simulink model "Controller_damping_cbf_22Franka"  (R2022b)
settings: Solver=FixedStepDiscrete  StartTime=0.0  StopTime=inf  FixedStep=0.001  RelTol=1e-3
PreLoadFcn:
  | set_param(gcs, 'RTWSystemTargetFile', 'franka_emika_panda.tlc');
  | 
  | demos_common_configs();
  | collision_behavior = ones(1,52)*100;
values from neighbouring files (symbols this model uses):
  b_sg = fliplr(B(end, :))    [init_damping_cbf.m]
  cbf_damping_params = [cbf_p_ths; cbf_v_ths; cbf_v_0; cbf_gamma; cbf_d_max;                        cbf_w_lin; cbf_w_quad; plane_normal; plane_offset;                        cbf_latch_entry; cbf_zone_hyst; cbf_latch_alpha; cbf_clip_drift;                        cbf_tau_rate; cbf_dt; cbf_gamma_pos_scale]    [init_damping_cbf.m]
  cbf_kappa = 0.85 * cbf_d_max / cbf_rho_eff    (= 82.6388888889)    [init_damping_cbf.m]
  cbf_stiff_decouple = 0    [init_damping_cbf.m]
  Dn = 20 * ones(7,1)    [init_damping_cbf.m]
  H_home = getTransform(Franka_robot, q_home, 'panda_link8', 'panda_link0')    [init_damping_cbf.m]
  Kn = 0 * ones(7,1)    [init_damping_cbf.m]
  plane_normal = [0.0; 0.0; 1.0]    [init_damping_cbf.m]
  q_home = q_init    [init_damping_cbf.m]
  q_init = [0 0  0  -(2/4)*pi  0  pi/2  -pi/4]'    [init_damping_cbf.m]
undefined symbols (not defined in the file or in its folder): DiscIntNeverNeededParam, Fext_mag
libraries: matrix_library x3, franka_simulink_library x2, Robotics_lib x1
(part 7 of 8)

== matlab function Controller_damping_cbf_22Franka/task space controller/Stiffnessforces/MATLAB Function3 ==
  data: H_I_t input; H_I_D input; Fk output; KdTrans input; KdRot input; Q_D_t output; x_tilde output
function [Fk, Q_D_t, x_tilde] = StiffnessVector(H_I_t, H_I_D, KdTrans, KdRot)

KdTrans = diag(KdTrans);
KdRot = diag(KdRot);

R_D_t = (H_I_D(1:3,1:3))'*H_I_t(1:3,1:3);

eta_D_t = 0.5*sqrt(abs(1+ R_D_t(1,1) +R_D_t(2,2) +R_D_t(3,3)));
epsi_D_t = 0.5.*[MySign(R_D_t(3,2) - R_D_t(2,3))*realsqrt(abs( R_D_t(1,1)-R_D_t(2,2)-R_D_t(3,3)+1));
                 MySign(R_D_t(1,3) - R_D_t(3,1))*realsqrt(abs(-R_D_t(1,1)+R_D_t(2,2)-R_D_t(3,3)+1));
                 MySign(R_D_t(2,1) - R_D_t(1,2))*realsqrt(abs(-R_D_t(1,1)-R_D_t(2,2)+R_D_t(3,3)+1))];
Q_D_t = [eta_D_t; epsi_D_t];

epsi_D_t_skew = [0,          -epsi_D_t(3), epsi_D_t(2);
                 epsi_D_t(3),    0,       -epsi_D_t(1);
                -epsi_D_t(2), epsi_D_t(1),       0]; 

x_tilde = H_I_t(1:3,4) - H_I_D(1:3,4);

Fktrans = KdTrans*x_tilde;
Fkrot = 2.*H_I_D(1:3,1:3)*(eta_D_t.*eye(3) + epsi_D_t_skew)*KdRot*epsi_D_t;

Fk = [Fktrans; Fkrot];

end

function x = MySign(val)
% modified sign-fuction, which returns
%                 { 1,  if x>=0
%   MySign(x) =   { -1, if x<0
% If one uses the classical sign function, i.e. sign(x) = 0 if x = 0, then
% an error occurs. This becomes clear if one used the rotation matrix 
% R = [0 1 0; 1 0 0; 0 0 -1]. Then the quaternion computation will return
% just zero elements. 
%
% Source: Robotics - Modelling, Planning and Control - Siciliano (2010)
% Chapter 2.6, page 54, equation (2.35)

x = 1;
if(val<0)
    x = -1;
end


end

== matlab function Controller_damping_cbf_22Franka/task space controller/Compute_F_nominal ==
  data: Fk input; F_nominal output; D0 input; V_tilde input; n_hp input; decouple input; massM input; lambdaM input; C input; Jg input; Jg_dot input; JgRightPseu input
function F_nominal = fcn(Fk, D0, V_tilde, n_hp, decouple, massM, lambdaM, C, Jg, Jg_dot, JgRightPseu)
massMInv = massM\eye(7);
massMInv = (massMInv + transpose(massMInv))./2;

F_lat = -Fk - D0*V_tilde;
if decouple > 0.5        % same decoupling as 'impedance controller1'
    n6 = n_hp(:)./norm(n_hp);
    Lambda_inv = Jg*massMInv*transpose(Jg);
    Lambda_inv = (Lambda_inv + transpose(Lambda_inv))./2;
    F_lat = F_lat - n6.*((transpose(n6)*Lambda_inv*F_lat)/(transpose(n6)*Lambda_inv*n6));
end

mu = lambdaM*(Jg*massMInv*C - Jg_dot);
F_nominal = F_lat - mu*JgRightPseu*V_tilde;   % spring + damping + uncompensated Cartesian Coriolis
end

== matlab function Controller_damping_cbf_22Franka/Franka Forward Dynamics /MATLAB Function ==
  data: wrench input; force output
function force = fcn(wrench)

force = wrench(1:3);

end

== matlab function Controller_damping_cbf_22Franka/MATLAB Function ==
  data: H input; p output
function p = fcn(H)

p = H(1:3,4);

== matlab function Controller_damping_cbf_22Franka/task space controller/MATLAB Function1 ==
  data: n_hp input; F_ext output; wrench_ext input
function F_ext = fcn(n_hp, wrench_ext)

% F_ext = (n_hp).*wrench_ext;
 F_ext = wrench_ext;
end

== matlab function Controller_damping_cbf_22Franka/task space controller/Compute eff d_max ==
  data: params_in input; params output; rho input; kappa input; d_max output
function [params, d_max] = fcn(params_in, rho, kappa)

params = params_in;
params(5) = min(params_in(5), kappa*rho); % d_max_eff
d_max = params(5);
end

== matlab function Controller_damping_cbf_22Franka/MATLAB Function2 ==
  data: H_init input; H_ref output; d input; R_I_t output
function [H_ref, R_I_t] = fcn(H_init, d)

H_ref = H_init;
% H_ref(1:3,4) = d;
R_I_t = H_ref(1:3,1:3);

end
